simulink model "Trayectory_Model"  (R2023b)
settings: Solver=VariableStepAuto  StartTime=0.0  StopTime=inf  RelTol=1e-3
PostLoadFcn:
  | % EICUSTOM_BINDING_BEGIN
  | eiCustomModelName=bdroot;
  | eiCustomProjectRoot=fileparts(get_param(eiCustomModelName,'FileName'));
  | while ~isfile(fullfile(eiCustomProjectRoot,'setup_custom_model.m'))
  |     eiCustomParent=fileparts(eiCustomProjectRoot);
  |     assert(~strcmp(eiCustomParent,eiCustomProjectRoot) && ~isempty(eiCustomParent),'EI:ProjectMissing','Keep this model inside the Edge Impulse project folder.');
  |     eiCustomProjectRoot=eiCustomParent;
  | end
  | addpath(eiCustomProjectRoot,'-begin');
  | ei_custom_model_binding('load',eiCustomModelName);
  | clear eiCustomModelName eiCustomProjectRoot eiCustomParent
  | % EICUSTOM_BINDING_END
InitFcn:
  | % EICUSTOM_BINDING_BEGIN
  | eiCustomModelName=bdroot;
  | eiCustomProjectRoot=fileparts(get_param(eiCustomModelName,'FileName'));
  | while ~isfile(fullfile(eiCustomProjectRoot,'setup_custom_model.m'))
  |     eiCustomParent=fileparts(eiCustomProjectRoot);
  |     assert(~strcmp(eiCustomParent,eiCustomProjectRoot) && ~isempty(eiCustomParent),'EI:ProjectMissing','Keep this model inside the Edge Impulse project folder.');
  |     eiCustomProjectRoot=eiCustomParent;
  | end
  | addpath(eiCustomProjectRoot,'-begin');
  | ei_custom_model_binding('refresh',eiCustomModelName);
  | clear eiCustomModelName eiCustomProjectRoot eiCustomParent
  | % EICUSTOM_BINDING_END
model workspace (MAT data in the model file):
  eiCustomBinding.includeDir = 'C:\Ago-Dic26\VSCode\Edge_Impules\Audrey_Lazara\EdgeImpulse_MATLAB_Integration\native'
  eiCustomBinding.importLibrary = 'C:\Ago-Dic26\VSCode\Edge_Impules\Audrey_Lazara\EdgeImpulse_MATLAB_Integration\build\eb16cb243767a9c4559b\cmake\lib\libei_inference_eb16cb243767a9c4559b.dll.a'
  eiCustomBinding.buildKey = 'eb16cb243767a9c4559b'
  eiCustomBinding.imageContract = [180 180 1]
undefined symbols (not defined in the file or in its folder): none, videoinput
libraries: imaqlib x1
settings Model: Creator=saray  LastModifiedBy=saray
settings SFSimCC: SimUserIncludeDirs="\"C:\\Ago-Dic26\\VSCode\\Edge_Impules\\Audrey_Lazara\\EdgeImpulse_MATLAB_Integration\\native\""  SimUserLibraries="\"C:\\Ago-Dic26\\VSCode\\Edge_Impules\\Audrey_Lazara\\EdgeImpulse_MATLAB_Integration\\build\\eb16cb243767a9c4559b\\cmake\\lib\\libei_inference_eb16cb243767a9c4559b.dll.a\""
settings SFSimCC: SimCustomHeaderCode=|
  | /* EICUSTOM_BINDING_BEGIN */
  | #include "ei_wrapper.h"
  | #include "mex.h"
  | /* EICUSTOM_BINDING_END */
settings SFSimCC: SimCustomInitializer=|
  | /* EICUSTOM_BINDING_BEGIN */
  | { int32_t ei_custom_status=ei_sim_start(5.000000000e-01f,0u,4096u,0u,0);
  | if(ei_custom_status<0) { char ei_custom_error[1024]; ei_get_last_error(ei_custom_error,1024);
  | mexErrMsgIdAndTxt("EI:SimInit","%s",ei_custom_error); } }
  | /* EICUSTOM_BINDING_END */
settings SFSimCC: SimCustomTerminator=|
  | /* EICUSTOM_BINDING_BEGIN */
  | ei_sim_stop();
  | /* EICUSTOM_BINDING_END */

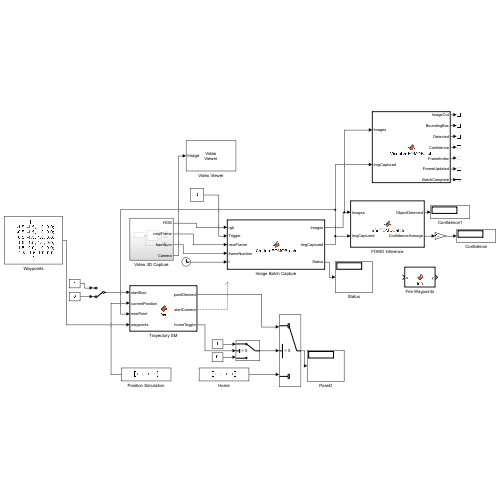
[thumbnail: Simulink's stored preview of the top-level diagram]
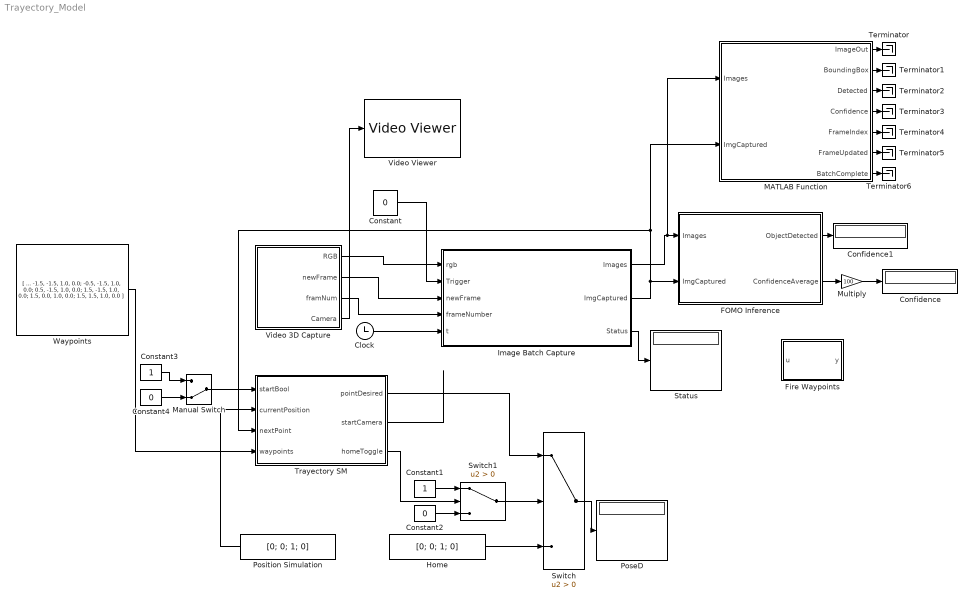
== system Trayectory_Model ==
  Clock : Clock
  Confidence : Display
  Confidence1 : Display
  Constant : Constant  Value=0  OutDataTypeStr=boolean
  Constant1 : Constant
  Constant2 : Constant  Value=0
  Constant3 : Constant
  Constant4 : Constant  Value=0
  FOMO Inference : MATLAB Function  TreatAsAtomicUnit=on
  Fire Waypoints : MATLAB Function  TreatAsAtomicUnit=on
  Home : Constant  Value=[0; 0; 1; 0]
  Image Batch Capture : MATLAB Function  TreatAsAtomicUnit=on
  MATLAB Function : MATLAB Function  TreatAsAtomicUnit=on
  Manual Switch : ManualSwitch  CurrentSetting=0
  Multiply : Gain  Gain=100
  PoseD : Display
  Position Simulation : Constant  Value=[0; 0; 1; 0]
  Status : Display
  Switch : Switch  Criteria=u2 > Threshold  SaturateOnIntegerOverflow=off  InputSameDT=off
  Switch1 : Switch  Criteria=u2 > Threshold  SaturateOnIntegerOverflow=off  InputSameDT=off
  Terminator{,1..6} (7 alike) : Terminator
  Trayectory SM : MATLAB Function  TreatAsAtomicUnit=on  SystemSampleTime=0.05
  Video 3D Capture : Subsystem
  Video Viewer : VideoViewer  FigPos=[1 862 1536 764]
  Waypoints : Constant  Value=|
      | [ ...
      |    -1.5, -1.5, 1.0, 0.0;
      |    -0.5, -1.5, 1.0, 0.0;
      |     0.5, -1.5, 1.0, 0.0;
      |     1.5, -1.5, 1.0, 0.0;
      |     1.5,  0.0, 1.0, 0.0;
      |     1.5,  1.5, 1.0, 0.0
      | ]
  wires:
  Home/1 -> Switch/3
  Switch1/1 -> Switch/2
  Trayectory SM/1(pointDesired) -> Switch/1
  Switch/1 -> PoseD/1
  Manual Switch/1 -> Trayectory SM/1(startBool)
  Position Simulation/1 -> Trayectory SM/2(currentPosition)
  Trayectory SM/2(startCamera) -> ?
  Trayectory SM/3(homeToggle) -> Switch1/2
  Constant1/1 -> Switch1/1
  Constant2/1 -> Switch1/3
  Constant4/1 -> Manual Switch/2
  Constant3/1 -> Manual Switch/1
  Image Batch Capture/3(Status) -> Status/1
  Video 3D Capture/1(RGB) -> Image Batch Capture/1(rgb)
  Video 3D Capture/2(newFrame) -> Image Batch Capture/3(newFrame)
  Video 3D Capture/3(framNum) -> Image Batch Capture/4(frameNumber)
  Clock/1 -> Image Batch Capture/5(t)
  Multiply/1 -> Confidence/1
  FOMO Inference/2(ConfidenceAverage) -> Multiply/1
  FOMO Inference/1(ObjectDetected) -> Confidence1/1
  Video 3D Capture/4(Camera) -> Video Viewer/1
  Image Batch Capture/2(ImgCaptured) -> MATLAB Function/2(ImgCaptured), Trayectory SM/3(nextPoint), FOMO Inference/2(ImgCaptured)
  Constant/1 -> Image Batch Capture/2(Trigger)
  Image Batch Capture/1(Images) -> MATLAB Function/1(Images), FOMO Inference/1(Images)
  MATLAB Function/1(ImageOut) -> Terminator/1
  MATLAB Function/2(BoundingBox) -> Terminator1/1
  MATLAB Function/4(Confidence) -> Terminator3/1
  MATLAB Function/3(Detected) -> Terminator2/1
  MATLAB Function/7(BatchComplete) -> Terminator6/1
  MATLAB Function/6(FrameUpdated) -> Terminator5/1
  MATLAB Function/5(FrameIndex) -> Terminator4/1
  Waypoints/1 -> Trayectory SM/4(waypoints)

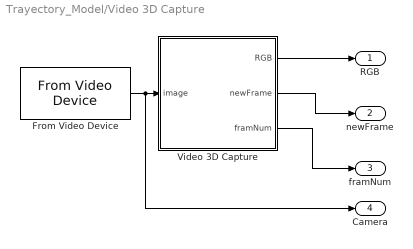
== system Trayectory_Model/Video 3D Capture ==
  From Video Device : imaqlib/From Video Device  DeviceMenu=winvideo 1 (HD Webcam)  Device=winvideo 1 (HD Webcam)  ObjConstructor=videoinput('winvideo', 1)  VideoFormatMenu=MJPG_1280x720  VideoFormat=MJPG_1280x720  VideoSource=input1  ROIPosition=[0 0 720 1280]  EnableHWTrigger=off  TriggerConfiguration=none/none  SampleTime=1/30  OutputPortsMode=One multidimensional signal  DataType=uint8  CanDoHWTrigger=no  ReturnedColorSpace=rgb  BlockHandle=698.0002  ROIWidth=1280  ROIHeight=720  ROIColumn=0  ROIRow=0  EngXMLPath=C:\Program Files\MATLAB\R2023b\toolbox\imaq\imaq\private  DevXMLPath=C:\ProgramData\MATLAB\SupportPackages\R2023b\toolbox\imaq\supportpackages\genericvideo\adaptor\win64  EngLibPath=C:\Program Files\MATLAB\R2023b\toolbox\imaq\imaqblks\imaqmex\win64  ColorSpace=rgb  BayerSensorAlignment=grbg  ImaqMode=off
  Video 3D Capture : MATLAB Function  TreatAsAtomicUnit=on
  RGB : Outport
  newFrame : Outport  Port=2
  framNum : Outport  Port=3
  Camera : Outport  Port=4
  wires:
  From Video Device/1 -> Camera/1, Video 3D Capture/1(image)
  Video 3D Capture/1(RGB) -> RGB/1
  Video 3D Capture/2(newFrame) -> newFrame/1
  Video 3D Capture/3(framNum) -> framNum/1

== matlab function Trayectory_Model/Image Batch Capture ==
  data: rgb input; Images output; Trigger input; newFrame input; frameNumber input; t input; ImgCaptured output; Status output
function [Images, ImgCaptured, Status] = CaptureFOMOBatch( ...
    rgb, Trigger, newFrame, frameNumber, t)
%#codegen
%
% Images:      uint8 [180 180 N]
% ImgCaptured: true only when the complete batch is available
%
% Status:
%   0 = idle
%   1 = capturing
%   2 = complete
%  -1 = invalid/backward clock
%  -2 = missing/late camera frame

% EDIT THESE BETWEEN SIMULATION RUNS:
N = 25;
CaptureSeconds = 3.0;

assert(N >= 1 && N == floor(N));
assert(isfinite(CaptureSeconds) && CaptureSeconds > 0);
assert(isa(rgb,'uint8') && isequal(size(rgb),[480 640 3]));
assert(islogical(Trigger) && isscalar(Trigger));
assert(islogical(newFrame) && isscalar(newFrame));
assert(isa(frameNumber,'uint64') && isscalar(frameNumber));
assert(isa(t,'double') && isscalar(t));

persistent bank ready active previous count startTime
persistent lastID haveID lastTime code

if isempty(previous)
    bank = zeros(180,180,N,'uint8');
    ready = false;
    active = false;
    previous = false;
    count = 0;
    startTime = 0;
    lastID = uint64(0);
    haveID = false;
    lastTime = 0;
    code = int32(0);
end

rising = Trigger && ~previous;
previous = Trigger;

% Invalid timing must never produce a completed batch.
if ~isfinite(t) || t < lastTime
    active = false;
    ready = false;
    code = int32(-1);

    Images = bank;
    ImgCaptured = ready;
    Status = code;
    return
end
lastTime = t;

% Accept a new request only when not already capturing.
if rising && ~active
    bank(:) = uint8(0);
    count = 0;
    ready = false;
    active = true;
    startTime = t;
    lastID = uint64(0);
    haveID = false;
    code = int32(1);
end

if active
    if N == 1
        interval = CaptureSeconds;
    else
        interval = CaptureSeconds / (N - 1);
    end

    % First target is at the trigger; last target is CaptureSeconds later.
    due = startTime + count*interval;

    % Permit camera timing quantization, but reject missed slots.
    maxLate = min(0.05, interval/2);

    if t > due + maxLate + 1e-9
        active = false;
        ready = false;
        code = int32(-2);

    elseif t + 1e-9 >= due && newFrame && ...
            (~haveID || frameNumber > lastID)

        k = count + 1;

        % Match the current project's squash + nearest-neighbor resize,
        % followed by grayscale conversion.
        for y = 1:180
            sy = floor((y - 0.5)*480/180) + 1;

            for x = 1:180
                sx = floor((x - 0.5)*640/180) + 1;

                value = 0.299*double(rgb(sy,sx,1)) ...
                      + 0.587*double(rgb(sy,sx,2)) ...
                      + 0.114*double(rgb(sy,sx,3));

                bank(y,x,k) = uint8(round(value));
            end
        end

        count = k;
        lastID = frameNumber;
        haveID = true;

        if count == N
            active = false;
            ready = true;
            code = int32(2);
        end
    end
end

Images = bank;
ImgCaptured = ready;
Status = code;
end

== matlab function Trayectory_Model/Trayectory SM ==
  data: startBool input; pointDesired output; currentPosition input; nextPoint input; startCamera output; homeToggle output; waypoints input

function [pointDesired, startCamera, homeToggle] = ...
    fcn(startBool, currentPosition, nextPoint,waypoints)
%#codegen
%
% SEQUENTIAL WAYPOINT STATE MACHINE
%
% Inputs:
%   startBool       : Boolean mission start signal
%   currentPosition : [X; Y; Z; Yaw] measured position (4x1)
%   nextPoint       : Boolean camera completion acknowledgment
%
% Outputs:
%   pointDesired    : [X; Y; 1; 0] desired reference (4x1)
%   startCamera     : Boolean camera activation
%   homeToggle      : Boolean mission-active output
%
% Operating principle:
%   1. Wait for startBool.
%   2. Command a waypoint.
%   3. Verify position stability for 3 seconds.
%   4. Activate the camera.
%   5. Wait for a fresh camera acknowledgment.
%   6. Advance or complete the mission.
%
% IMPORTANT:
%   Execute this block at a discrete sample time of 0.05 s.

%% =========================================================
%  1. USER CONFIGURATION
% ==========================================================

% Fixed sample time and verification duration
Ts = 0.05;                 % Seconds
settlingTime = 3.0;        % Seconds
windowSize = 60;           % settlingTime / Ts

% Workspace boundaries (meters)
xMin = -1.5;
xMax =  1.5;
yMin = -1.5;
yMax =  1.5;

% Constant altitude and yaw references
zDesired = 1.0;
yawDesired = 0.0;          % Radians

% Mean-position tolerances
tolMean = [ ...
    0.10;                  % X error (m)
    0.10;                  % Y error (m)
    0.10;                  % Z error (m)
    5.0*pi/180 ];          % Yaw error (rad)

% Instantaneous stabilization tolerances
% Every sample in the verification window must
% remain within these limits.
tolInstant = [ ...
    0.15;                  % X error (m)
    0.15;                  % Y error (m)
    0.15;                  % Z error (m)
    8.0*pi/180 ];          % Yaw error (rad)

%% =========================================================
%  2. HARD-CODED WAYPOINTS
% ==========================================================

% Each row is [X, Y, Z, Yaw].
%
% EDIT THESE POINTS TO DEFINE THE FINAL MISSION.
% All X,Y coordinates must be within [-1.5, 1.5].
%
% These coordinates are examples.

% waypoints = [ ...
%    -1.5, -1.5, 1.0, 0.0;
%    -0.5, -1.5, 1.0, 0.0;
%     0.5, -1.5, 1.0, 0.0;
%     1.5, -1.5, 1.0, 0.0;
%     1.5,  0.0, 1.0, 0.0;
%     1.5,  1.5, 1.0, 0.0
% ];

numberOfWaypoints = size(waypoints, 1);

%% =========================================================
%  3. STATE DEFINITIONS
% ==========================================================

STATE_IDLE     = uint8(0);
STATE_MOVE     = uint8(1);
STATE_VERIFY   = uint8(2);
STATE_CAMERA   = uint8(3);
STATE_ADVANCE  = uint8(4);
STATE_COMPLETE = uint8(5);

%% =========================================================
%  4. PERSISTENT STATE VARIABLES
% ==========================================================

persistent state
persistent waypointIndex

% Position verification memory
persistent errorHistory
persistent errorSum
persistent sampleCount
persistent writeIndex

% Camera handshake memory
persistent cameraArmed

if isempty(state)

    state = STATE_IDLE;
    waypointIndex = 1;

    % Fixed-size circular buffer
    errorHistory = zeros(4, windowSize);
    errorSum = zeros(4,1);

    sampleCount = 0;
    writeIndex = 1;

    cameraArmed = false;

end

%% =========================================================
%  5. DEFAULT OUTPUTS
% ==========================================================

startCamera = false;
homeToggle = true;

% Validate position feedback before using it.
validFeedback = all(isfinite(currentPosition));

% Default command before mission start.
% Hold measured XY, with fixed Z and yaw.
if validFeedback
    pointDesired = [ ...
        currentPosition(1);
        currentPosition(2);
        zDesired;
        yawDesired ];
else
    pointDesired = [0.0; 0.0; zDesired; yawDesired];
end

% Restrict initial references to the workspace.
pointDesired(1) = min(max(pointDesired(1), xMin), xMax);
pointDesired(2) = min(max(pointDesired(2), yMin), yMax);

% Once started, always command the stored waypoint.
if state ~= STATE_IDLE

    pointDesired = waypoints(waypointIndex, :).';

    % Enforce workspace restrictions.
    pointDesired(1) = min(max(pointDesired(1), xMin), xMax);
    pointDesired(2) = min(max(pointDesired(2), yMin), yMax);

    % Enforce constant altitude and yaw.
    pointDesired(3) = zDesired;
    pointDesired(4) = yawDesired;

end

%% =========================================================
%  6. POSITION ERROR CALCULATION
% ==========================================================

positionError = zeros(4,1);

if validFeedback

    positionError(1) = ...
        currentPosition(1) - pointDesired(1);

    positionError(2) = ...
        currentPosition(2) - pointDesired(2);

    positionError(3) = ...
        currentPosition(3) - pointDesired(3);

    % Wrapped yaw error in [-pi, pi].
    yawError = currentPosition(4) - pointDesired(4);

    positionError(4) = atan2( ...
        sin(yawError), cos(yawError));

end

% Instantaneous position convergence condition.
insideTolerance = false;

if validFeedback

    insideTolerance = ...
        all(abs(positionError) <= tolInstant);

end

%% =========================================================
%  7. FINITE-STATE MACHINE
% ==========================================================

switch state

    %% -----------------------------------------------------
    %  STATE 0: IDLE
    % ------------------------------------------------------

    case STATE_IDLE

        startCamera = false;
        homeToggle = true;

        if startBool

            waypointIndex = 1;

            % Reset verification memory.
            errorHistory(:) = 0.0;
            errorSum(:) = 0.0;

            sampleCount = 0;
            writeIndex = 1;

            % Reset camera handshake.
            cameraArmed = false;

            state = STATE_MOVE;

        end

    %% -----------------------------------------------------
    %  STATE 1: MOVE TO WAYPOINT
    % ------------------------------------------------------

    case STATE_MOVE

        startCamera = false;
        homeToggle = true;

        if insideTolerance

            % Enter stabilization verification.
            errorHistory(:) = 0.0;
            errorSum(:) = 0.0;

            sampleCount = 0;
            writeIndex = 1;

            state = STATE_VERIFY;

        end

    %% -----------------------------------------------------
    %  STATE 2: VERIFY POSITION STABILITY
    % ------------------------------------------------------

    case STATE_VERIFY

        startCamera = false;
        homeToggle = true;

        if ~insideTolerance

            % Device left stabilization region or
            % feedback became invalid.
            %
            % Discard all previous verification samples.

            errorHistory(:) = 0.0;
            errorSum(:) = 0.0;

            sampleCount = 0;
            writeIndex = 1;

            state = STATE_MOVE;

        else

            % Add current error to the rolling window.
            if sampleCount < windowSize

                % Window not full yet.
                errorHistory(:, writeIndex) = positionError;

                errorSum = errorSum + positionError;

                sampleCount = sampleCount + 1;

            else

                % Remove oldest sample, insert newest.
                oldestError = errorHistory(:, writeIndex);

                errorSum = errorSum - oldestError;

                errorHistory(:, writeIndex) = positionError;

                errorSum = errorSum + positionError;

            end

            % Advance circular buffer index.
            writeIndex = writeIndex + 1;

            if writeIndex > windowSize
                writeIndex = 1;
            end

            % Evaluate convergence after 3 full seconds.
            if sampleCount >= windowSize

                meanError = errorSum / double(windowSize);

                meanConverged = ...
                    all(abs(meanError) <= tolMean);

                if meanConverged

                    % The waypoint is stable.
                    % Begin a new camera capture cycle.

                    cameraArmed = false;

                    state = STATE_CAMERA;

                end

            end

        end

    %% -----------------------------------------------------
    %  STATE 3: CAMERA ACQUISITION
    % ------------------------------------------------------

    case STATE_CAMERA

        startCamera = true;
        homeToggle = true;

        % Handshake protocol:
        %
        % A low camera-completion signal must first
        % be observed during this capture state.
        %
        % Only a subsequent high signal is accepted.
        %
        % This prevents a previous camera acknowledgment
        % from being reused for a new waypoint.

        if ~nextPoint

            % Camera completion is low.
            % Arm acceptance of a fresh acknowledgment.
            cameraArmed = true;

        elseif cameraArmed

            % Camera has completed the current capture.
            % Accept exactly one acknowledgment.

            cameraArmed = false;

            startCamera = false;

            state = STATE_ADVANCE;

        end

    %% -----------------------------------------------------
    %  STATE 4: ADVANCE WAYPOINT
    % ------------------------------------------------------

    case STATE_ADVANCE

        % Handled by the post-switch advancement logic.

    %% -----------------------------------------------------
    %  STATE 5: MISSION COMPLETE
    % ------------------------------------------------------

    case STATE_COMPLETE

        startCamera = false;
        homeToggle = false;

    otherwise

        % Fail-safe internal state recovery.
        % Do not automatically restart the mission.

        state = STATE_COMPLETE;

end

%% =========================================================
%  8. WAYPOINT ADVANCEMENT / TERMINATION
% ==========================================================

% This section also executes immediately after a camera
% acknowledgment sets STATE_ADVANCE, so no extra
% simulation step is required for mission completion.

if state == STATE_ADVANCE

    startCamera = false;

    % Clear verification memory before the next waypoint.
    errorHistory(:) = 0.0;
    errorSum(:) = 0.0;

    sampleCount = 0;
    writeIndex = 1;

    cameraArmed = false;

    if waypointIndex < numberOfWaypoints

        % Advance exactly one waypoint.
        waypointIndex = waypointIndex + 1;

        state = STATE_MOVE;

    else

        % Final waypoint was photographed.
        % Mission is now permanently complete.

        state = STATE_COMPLETE;

    end

end

%% =========================================================
%  9. FINAL OUTPUT ASSIGNMENT
% ==========================================================

if state ~= STATE_IDLE

    % Command the active waypoint, including updates
    % after state advancement.
    pointDesired = waypoints(waypointIndex, :).';

    % Hard workspace constraints.
    pointDesired(1) = min(max(pointDesired(1), xMin), xMax);
    pointDesired(2) = min(max(pointDesired(2), yMin), yMax);

    pointDesired(3) = zDesired;
    pointDesired(4) = yawDesired;

end

% Outputs are defined by the final active state.
startCamera = (state == STATE_CAMERA);

if state == STATE_COMPLETE

    homeToggle = false;

else

    homeToggle = true;

end

end

== matlab function Trayectory_Model/Video 3D Capture/Video 3D Capture ==
  data: RGB output; newFrame output; framNum output; image input
function [RGB, newFrame, framNum] = VideoDeviceToQUARC(image)
%#codegen
%
% INPUT:
%   image: fixed-size uint8 [H W 3].
%   H and W are inherited from the connected acquisition block.
%
% OUTPUTS:
%   RGB:      uint8 [480 640 3]
%   newFrame: logical scalar
%   framNum:  uint64 scalar
%
% Execute at the acquisition rate, 1/30 second.
% Enable Read All Frames on From Video Device.
%
% newFrame assumes one newly delivered acquisition per execution.
% framNum is a software counter, not a hardware frame identifier.

assert(isa(image,'uint8') && isreal(image), ...
    'Input must be a real uint8 RGB image.');

assert(ndims(image)==3 && size(image,3)==3, ...
    'Connect one H-by-W-by-3 RGB signal, not separate color planes.');

assert(size(image,1)>0 && size(image,2)>0, ...
    'Input image must not be empty.');

sourceHeight = double(size(image,1));
sourceWidth  = double(size(image,2));

% false: resize the entire image, allowing aspect-ratio distortion.
% true: center-crop to 4:3 before resizing, preserving proportions.
CENTER_CROP = false;

cropHeight = sourceHeight;
cropWidth  = sourceWidth;
topOffset  = 0;
leftOffset = 0;

if CENTER_CROP
    if sourceWidth*480 > sourceHeight*640
        % Input is wider than the required 4:3 output.
        cropWidth = min(sourceWidth, ...
            max(1,floor(sourceHeight*640/480)));

        leftOffset = floor((sourceWidth-cropWidth)/2);
    else
        % Input is taller than the required 4:3 output.
        cropHeight = min(sourceHeight, ...
            max(1,floor(sourceWidth*480/640)));

        topOffset = floor((sourceHeight-cropHeight)/2);
    end
end

% Fixed-length indices ensure a fixed 480x640 output.
rows = topOffset ...
     + floor(((0:479)+0.5)*(cropHeight/480)) + 1;

cols = leftOffset ...
     + floor(((0:639)+0.5)*(cropWidth/640)) + 1;

% Explicitly protect array boundaries.
rows = min(sourceHeight,max(1,rows));
cols = min(sourceWidth,max(1,cols));

% Preserve RGB channels and uint8 data type.
RGB = image(rows,cols,:);

persistent counter

if isempty(counter)
    counter = uint64(0);
end

assert(counter<intmax('uint64'), ...
    'Frame counter exhausted; restart simulation.');

counter = counter+uint64(1);

framNum = counter;
newFrame = true;
end

== matlab function Trayectory_Model/FOMO Inference ==
  data: Images input; ObjectDetected output; ImgCaptured input; ConfidenceAverage output
function [ObjectDetected, ConfidenceAverage] = InferFOMOBatch(Images, ImgCaptured)
%#codegen
%
% INPUTS:
% Images       : Fixed-size uint8 [180 180 N], from CaptureFOMOBatch.
% ImgCaptured  : Logical scalar, from CaptureFOMOBatch.
%
% OUTPUTS:
% ObjectDetected    : Logical; true when MORE THAN HALF the images detect Fire.
% ConfidenceAverage : Double [0,1], rounded to two decimal places.
%
% AVERAGING POLICY:
% Each image uses the project's existing confidence threshold and
% highest-confidence detection selection. No detection contributes zero.
% ConfidenceAverage averages over ALL N images, including those zeros.
% It represents mean detection confidence, not classification accuracy.
%
% EXECUTION:
% A rising ImgCaptured edge accepts one complete batch.
% The batch is copied once to protect it from subsequent input changes.
% One image is processed per block execution while simulation is running.
% After N executions, both outputs update and remain held.
% A continuously high ImgCaptured signal never repeats the batch.
% Outputs are false/0 initially and while processing a newly accepted batch.
%
% REQUIRED MODEL SETUP -- MATLAB Command Window, before simulation:
%   setup_project(false);
%   build_model();
%   configure_simulink_model('YourModelName');
%
% The helper changes solver/sample-time settings. Restore the settings
% required by your QUARC model afterwards. Execute this block at a
% discrete sample time, for example the camera's sample time.
%
% Model custom initialization/termination loads/releases the native engine
% once per simulation. Initialization is NOT repeated for each image.
% Each native inference is synchronous and blocks its current execution;
% this is not an asynchronous worker or a hard real-time guarantee.
%
% The existing DLL supports Windows x64. Other QUARC targets require
% a compatible native backend and target-specific linking.
%
% Keep runtime assertions enabled. Native errors or overlapping batches
% stop simulation instead of being silently interpreted as "no detection".
% Use one instance with exclusive access to the inference engine.
%
% Compiled and tested in MATLAB R2023b/Simulink using the existing bridge,
% synthetic detection batches, and the actual Fire model.
% Physical QUARC target execution has not been verified.

assert(isa(Images,'uint8') && isreal(Images));
assert(ndims(Images)<=3 && size(Images,1)==180 && size(Images,2)==180);
assert(islogical(ImgCaptured) && isscalar(ImgCaptured));

N = size(Images,3);
assert(N >= 1);

coder.cinclude('ei_wrapper.h');

persistent batch processing previousReady nextImage positiveCount
persistent sumPercent heldDecision heldAverage lastResultID

if isempty(previousReady)
    batch = zeros(180,180,N,'uint8');
    processing = false;
    previousReady = false;
    nextImage = 1;
    positiveCount = 0;
    sumPercent = 0.0;
    heldDecision = false;
    heldAverage = 0.0;
    lastResultID = uint64(0);
end

% Accept each completed capture exactly once.
newBatch = ImgCaptured && ~previousReady;
previousReady = ImgCaptured;

overlap = newBatch && processing;

if overlap
    processing = false;
    heldDecision = false;
    heldAverage = 0.0;
end

assert(~overlap, ...
    'Previous batch is still processing. Wait before submitting another completed batch.');

if newBatch && ~overlap
    batch = Images;

    nextImage = 1;
    positiveCount = 0;
    sumPercent = 0.0;

    heldDecision = false;
    heldAverage = 0.0;
    processing = true;
end

% Process one snapshot image per simulation execution.
if processing
    image = batch(:,:,nextImage);

    percent = single(0);
    objectClass = uint8(0);
    detected = uint8(0);
    resultID = uint64(0);
    nativeStatus = int32(0);

    nativeStatus = coder.ceval( ...
        'ei_sim_infer', ...
        coder.rref(image), ...
        uint64(numel(image)), ...
        uint32(size(image,1)), ...
        uint32(size(image,2)), ...
        coder.wref(percent), ...
        coder.wref(objectClass), ...
        coder.wref(detected), ...
        coder.wref(resultID));

    % Status 1 = valid detection; status 2 = successful no-detection.
    % Increasing result IDs also prevent accepting stale native results.
    valid = isfinite(percent) && percent>=0 && percent<=100 ...
        && resultID>lastResultID ...
        && ((nativeStatus==int32(1) && detected==uint8(1)) ...
        ||  (nativeStatus==int32(2) && detected==uint8(0)));

    if ~valid
        processing = false;
        heldDecision = false;
        heldAverage = 0.0;
    end

    assert(valid, ...
        'Native FOMO inference failed. Check DLL initialization, ownership, dimensions and native status.');

    if valid
        lastResultID = resultID;

        if detected~=0
            positiveCount = positiveCount + 1;
            sumPercent = sumPercent + double(percent);
        end

        if nextImage == N
            % Strict majority; an exact tie returns false.
            heldDecision = positiveCount > double(N)/2.0;

            % Convert percent to [0,1], averaging across all N images.
            meanConfidence = sumPercent/(100.0*double(N));
            meanConfidence = min(1.0,max(0.0,meanConfidence));

            heldAverage = round(100.0*meanConfidence)/100.0;
            processing = false;
        else
            nextImage = nextImage + 1;
        end
    end
end

ObjectDetected = heldDecision;
ConfidenceAverage = heldAverage;
end

== matlab function Trayectory_Model/MATLAB Function ==
  data: Images input; ImageOut output; ImgCaptured input; BoundingBox output; Detected output; Confidence output; FrameIndex output; FrameUpdated output; BatchComplete output
function [ImageOut, BoundingBox, Detected, Confidence, FrameIndex, ...
          FrameUpdated, BatchComplete] = VisualizeFOMOBatch(Images, ImgCaptured)
%#codegen
% Images: fixed-size uint8 [180 180 N], currently N=20.
% ImgCaptured: logical scalar; rising edge accepts a complete batch.
%
% ImageOut: exact original uint8 [180 180] grayscale frame.
% BoundingBox: uint32 [x y width height], native ZERO-BASED coordinates.
% Detected: logical detection flag for the current image.
% Confidence: single [0,1], individual image confidence.
% FrameIndex: uint32 index 1..N, initially zero.
% FrameUpdated: one-execution pulse for each processed image.
% BatchComplete: latched true after N images, reset by the next batch.
%
% One inference and one figure update per execution.
% Figures are reused by image index across batches.
% Requires setup_fomo_visualization and existing model initialization.

coder.extrinsic('ei_visualization_step');

assert(~coder.target('Rtw'), ...
    'This viewer requires MATLAB normal simulation.');
assert(isa(Images,'uint8') && isreal(Images));
assert(ndims(Images)<=3 && ...
    size(Images,1)==180 && size(Images,2)==180);
assert(islogical(ImgCaptured) && isscalar(ImgCaptured));

N = size(Images,3);
assert(N>=1 && N<=double(intmax('uint32')));

persistent bank busy previousReady nextIndex batchID lastID
persistent heldImage heldBox heldDetected heldConfidence heldIndex complete

if isempty(previousReady)
    bank = zeros(180,180,N,'uint8');
    busy = false;
    previousReady = false;
    nextIndex = 1;
    batchID = uint64(0);
    lastID = uint64(0);

    heldImage = zeros(180,180,'uint8');
    heldBox = zeros(1,4,'uint32');
    heldDetected = false;
    heldConfidence = single(0);
    heldIndex = uint32(0);
    complete = false;
end

FrameUpdated = false;

newBatch = ImgCaptured && ~previousReady;
previousReady = ImgCaptured;

assert(~(newBatch && busy), ...
    'Visualization is still processing the preceding batch.');

if newBatch
    assert(batchID<intmax('uint64'), ...
        'Restart simulation: batch counter exhausted.');

    % Snapshot protects images from subsequent capture updates.
    bank = Images;
    nextIndex = 1;
    batchID = batchID + uint64(1);
    complete = false;
    busy = true;

    heldImage(:) = uint8(0);
    heldBox(:) = uint32(0);
    heldDetected = false;
    heldConfidence = single(0);
    heldIndex = uint32(0);
end

if busy
    frame = bank(:,:,nextIndex);

    % Explicit types/sizes are required for extrinsic outputs.
    box = zeros(1,4,'uint32');
    found = false;
    score = single(0);
    nativeID = uint64(0);

    [box, found, score, nativeID] = ei_visualization_step( ...
        frame, uint32(nextIndex), uint32(N), batchID);

    assert(nativeID>lastID && ...
        isfinite(score) && score>=0 && score<=1, ...
        'Invalid or stale visualization inference result.');

    lastID = nativeID;

    % The rectangle is a figure overlay; these pixels stay unchanged.
    heldImage = frame;
    heldBox = box;
    heldDetected = found;
    heldConfidence = score;
    heldIndex = uint32(nextIndex);
    FrameUpdated = true;

    if nextIndex==N
        complete = true;
        busy = false;
    else
        nextIndex = nextIndex + 1;
    end
end

ImageOut = heldImage;
BoundingBox = heldBox;
Detected = heldDetected;
Confidence = heldConfidence;
FrameIndex = heldIndex;
BatchComplete = complete;
end

== matlab function Trayectory_Model/Fire Waypoints ==
  data: u input; y output
function y = fcn(u)

y = u;
